simulink model "Part1_2024b"  (R2024b)
settings: Solver=VariableStepAuto  StartTime=0.0  StopTime=20  RelTol=1e-3
values from neighbouring files (symbols this model uses):
  A_full = [   0,                           1,                         0,       0 ... (first row only)    [Part1_Part2_script.m]
  B_full = [           0,               0 ... (first row only)    [Part1_Part2_script.m]
  C_speed = minreal( (1/Gz_motor) * (F_star / (1 - F_star)) )    [Part1_Part2_script.m]
  Kp = 0.77    [Part1_Part2_script.m]
  Ts = (2*pi) / (20 * wspeed_loop)    (= 0.0628318530718)    [Part1_Part2_script.m]
undefined symbols (not defined in the file or in its folder): dspblkCoreblockFVToolHelper, gcbh
settings Model: Creator=karimdoubie  LastModifiedBy=Riccardo
settings ConfigComp: CovBoundaryAbsTol=1.0e-5

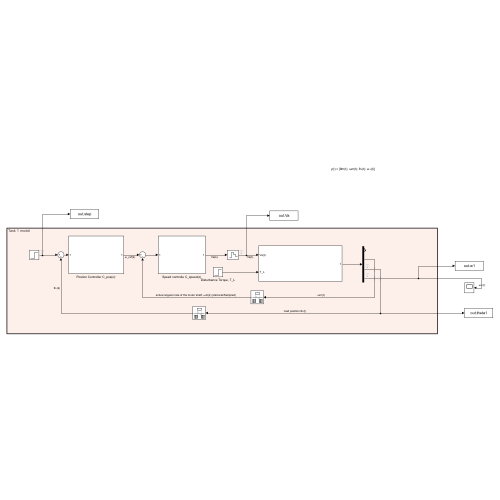
[thumbnail: Simulink's stored preview of the top-level diagram]
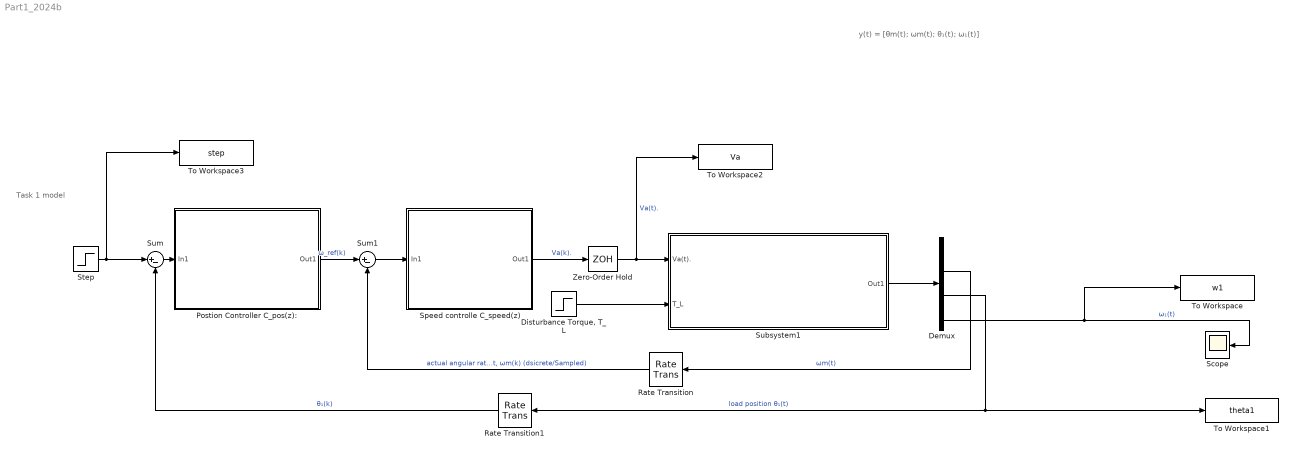
== system Part1_2024b ==
  note: y(t) = [θm(t); ωm(t); θ₁(t); ω₁(t)]
  note: Task 1 model
  Demux : Demux
  "Disturbance Torque, T_L" : Step  Time=6  After=0.05  SampleTime=0
  Postion Controller C_pos(z): : Subsystem
  Rate Transition : RateTransition  OutPortSampleTime=Ts
  Rate Transition1 : RateTransition  OutPortSampleTime=Ts
  Scope : Scope
  Speed controlle C_speed(z) : Subsystem
  Step : Step  Time=2  After=deg2rad(60)  SampleTime=0
  Subsystem1 : Subsystem
  Sum : Sum  Inputs=|+-
  Sum1 : Sum  Inputs=|+-
  To Workspace : ToWorkspace  VariableName=w1  SaveFormat=Timeseries  SampleTime=-1
  To Workspace1 : ToWorkspace  VariableName=theta1  SaveFormat=Timeseries  SampleTime=-1
  To Workspace2 : ToWorkspace  VariableName=Va  SaveFormat=Timeseries  SampleTime=-1
  To Workspace3 : ToWorkspace  VariableName=step  SaveFormat=Timeseries  SampleTime=-1
  Zero-Order Hold : ZeroOrderHold  SampleTime=Ts
  wires:
  Demux/3 -> To Workspace1/1, Rate Transition1/1  "load position θ₁(t)"
  Sum1/1 -> Speed controlle C_speed(z)/1(In1)
  Rate Transition1/1 -> Sum/2  "θ₁(k)"
  Rate Transition/1 -> Sum1/2  "actual angular rate of the motor shaft, ωm(k) (dsicrete/Sampled)"
  "Disturbance Torque, T_L"/1 -> Subsystem1/2(T_L)
  Step/1 -> Sum/1, To Workspace3/1
  Sum/1 -> Postion Controller C_pos(z):/1(In1)
  Demux/2 -> Rate Transition/1  "ωm(t)"
  Zero-Order Hold/1 -> Subsystem1/1(Va(t).), To Workspace2/1  "Va(t)."
  Postion Controller C_pos(z):/1(Out1) -> Sum1/1  "ω_ref(k)"
  Speed controlle C_speed(z)/1(Out1) -> Zero-Order Hold/1  "Va(k)."
  Subsystem1/1(Out1) -> Demux/1
  Demux/4 -> To Workspace/1, Scope/1  "ω₁(t)"

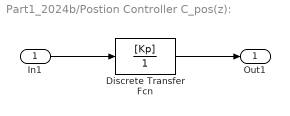
== system Part1_2024b/Postion Controller C_pos(z): ==
  In1 : Inport
  Discrete Transfer Fcn : DiscreteTransferFcn  LoadFcn=dspblkCoreblockFVToolHelper(gcbh,'load');  Numerator=[Kp]  Denominator=[1]
      settings: CopyFcn=dspblkCoreblockFVToolHelper(gcbh,'copy');  DeleteFcn=dspblkCoreblockFVToolHelper(gcbh,'close');  ModelCloseFcn=dspblkCoreblockFVToolHelper(gcbh,'close');  PreSaveFcn=dspblkCoreblockFVToolHelper(gcbh,'presave');  PostSaveFcn=dspblkCoreblockFVToolHelper(gcbh,'postsave');  CloseFcn=dspblkCoreblockFVToolHelper(gcbh,'close');
  Out1 : Outport
  wires:
  In1/1 -> Discrete Transfer Fcn/1
  Discrete Transfer Fcn/1 -> Out1/1

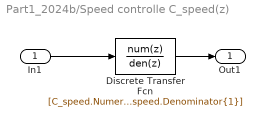
== system Part1_2024b/Speed controlle C_speed(z) ==
  In1 : Inport
  Discrete Transfer Fcn : DiscreteTransferFcn  LoadFcn=dspblkCoreblockFVToolHelper(gcbh,'load');  Numerator=[C_speed.Numerator{1}]  Denominator=[C_speed.Denominator{1}]
      settings: CopyFcn=dspblkCoreblockFVToolHelper(gcbh,'copy');  DeleteFcn=dspblkCoreblockFVToolHelper(gcbh,'close');  ModelCloseFcn=dspblkCoreblockFVToolHelper(gcbh,'close');  PreSaveFcn=dspblkCoreblockFVToolHelper(gcbh,'presave');  PostSaveFcn=dspblkCoreblockFVToolHelper(gcbh,'postsave');  CloseFcn=dspblkCoreblockFVToolHelper(gcbh,'close');
  Out1 : Outport
  wires:
  Discrete Transfer Fcn/1 -> Out1/1
  In1/1 -> Discrete Transfer Fcn/1

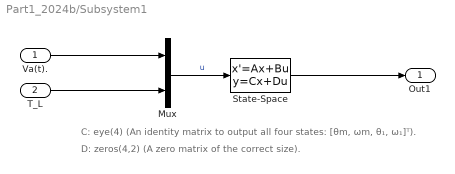
== system Part1_2024b/Subsystem1 ==
  note: D: zeros(4,2) (A zero matrix of the correct size).
  note: C: eye(4) (An identity matrix to output all four states: [θm, ωm, θ₁, ω₁]ᵀ).
  Va(t). : Inport
  T_L : Inport  Port=2
  Mux : Mux  Inputs=2
  State-Space : StateSpace  A=A_full  B=B_full  C=eye(4)  D=zeros(4,2)  InitialCondition=0
  Out1 : Outport
  wires:
  State-Space/1 -> Out1/1
  T_L/1 -> Mux/2
  Va(t)./1 -> Mux/1
  Mux/1 -> State-Space/1  "u"
